simulink model "proposed"  (R2024b)
settings: Solver=VariableStepAuto  StartTime=0.0  StopTime=10  RelTol=1e-3
undefined symbols (not defined in the file or in its folder): G, Initial_level, IR, Qin_L, Qout_L, SA_U, TE, Temp, Water_Const, WD
libraries: spsVoltageMeasurementLib x10, spsSeriesRLCBranchLib x5, spsGroundLib x4, spsIGBTDiodeLib x4, simulink x3, spsThreePhaseParallelRLCLoadLib x2, spsCurrentMeasurementLib x2, spsPVArrayLib x2, spspowerguiLib x2, spsThreePhaseSourceLib x1, spsExcitationSystemLib x1, spsHydraulicTurbineandGovernorLib x1
settings Model: Creator=skill  LastModifiedBy=skill
settings DataIOCC: ReturnWorkspaceOutputs=off
settings OptimizationCC: DefaultUnderspecifiedDataType=single

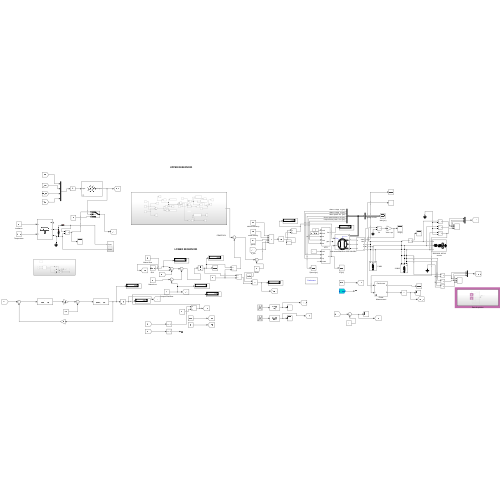
[thumbnail: Simulink's stored preview of the top-level diagram]
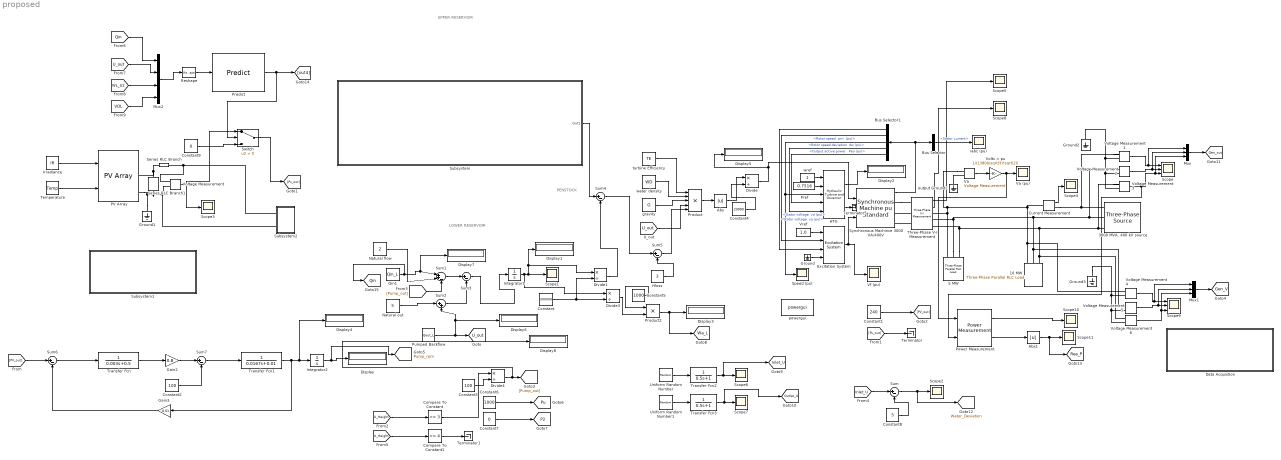
== system proposed ==
  note: UPPER RESERVOIR
  note: PENSTOCK
  note: LOWER RESERVOIR
  " Iabc (pu)" : Scope
  " Speed (pu)" : Scope
  10 MW : spsThreePhaseParallelRLCLoadLib/Three-Phase Parallel RLC Load  LConnTagsString=A|B|C  Configuration=Y (grounded)  NominalVoltage=400  Vabc=[1e3 1e3 1e3]  Vabcp=[1e3 1e3 1e3]  NominalFrequency=50  UnbalancedPower=off  ActivePower=360  InductivePower=0  CapacitivePower=0  Pabc=[10e3 9e3 11e3]  QLabc=[100 90 110]  QCabc=[100 90 110]  Pabcp=[10e3 9e3 11e3]  QLabcp=[100 90 110]  QCabcp=[100 90 110]  Measurements=None  LoadType=constant Z
  "3000 MVA, 400 kV source" : spsThreePhaseSourceLib/Three-Phase Source  InternalConnection=Yg  VoltagePhases=off  Voltage=400  PhaseAngle=0  Voltage_phases=[25e3 25e3 25e3]/sqrt(3)  PhaseAngles_phases=[0 -120 +120]  Frequency=50  NonIdealSource=on  SpecifyImpedance=on  Resistance=0.529  Inductance=0.0140  ShortCircuitLevel=3000  BaseVoltage=400  XRratio=10  BusType=swing  Pref=10e3  Qref=0  Prefabc=[10e3, 10e3, 10e3]  Qrefabc=[0, 0, 0]  Qmin=-inf  Qmax=inf
  5 MW : spsThreePhaseParallelRLCLoadLib/Three-Phase Parallel RLC Load  LConnTagsString=A|B|C  Configuration=Y (grounded)  NominalVoltage=380  Vabc=[1e3 1e3 1e3]  Vabcp=[1e3 1e3 1e3]  NominalFrequency=50  UnbalancedPower=off  ActivePower=200  InductivePower=0  CapacitivePower=0  Pabc=[10e3 9e3 11e3]  QLabc=[100 90 110]  QCabc=[100 90 110]  Pabcp=[10e3 9e3 11e3]  QLabcp=[100 90 110]  QCabcp=[100 90 110]  Measurements=None  LoadType=constant Z
  Abs : Abs  SaturateOnIntegerOverflow=off
  Abs1 : Abs  SaturateOnIntegerOverflow=off
  Bus Selector : BusSelector  OutputSignals=Stator current
  Bus Selector1 : BusSelector  OutputSignals="dq0 components.Stator voltage  vq (pu),dq0 components.Stator voltage  vd (pu),Mechanical.Rotor speed  wm  (pu),Mechanical.Rotor speed deviation  dw (pu),Output active power   Peo (pu)"
  Compare To Constant : simulink/Logic and Bit Operations/Compare To Constant  relop=<=  const=3  OutDataTypeStr=boolean
  Compare To Constant1 : simulink/Logic and Bit Operations/Compare To Constant  relop=>=  const=4  OutDataTypeStr=boolean
  Constant : Constant  Value=300000
  Constant1 : Constant  Value=240
  Constant2 : Constant  Value=100
  Constant3 : Constant  Value=100
  Constant4 : Constant  Value=23000
  Constant5 : Constant  Value=1000
  Constant6 : Constant  Value=1000
  Constant7 : Constant  Value=0
  Constant8 : Constant  Value=5
  Constant9 : Constant  Value=0
  Current Measurement : spsCurrentMeasurementLib/Current Measurement  PhasorSimulation=off  OutputType=Complex  PSBequivalent=0
  Data Acquistion : Subsystem
  Display{,1..8} (9 alike) : Display
  Divide{,1,3..4} (4 alike) : Product  Inputs=*/
  Excitation System : spsExcitationSystemLib/Excitation System  tr=20e-3  reg=[ 300, 0.001 ]  exc=[ 1, 0 ]  tgr=[ 0, 0 ]  damp=[ 0.001, 0.1 ]  sat=[ 0, 0 ]  lim=[ -11.5, 11.5, 0 ]  v0=[1,1.0]
  Gain2 : Gain  Gain=0.8
  Gain3 : Gain  Gain=0.01
  Ground : Ground
  Ground1 : spsGroundLib/Ground  LConnTagsString=a
  Ground2 : spsGroundLib/Ground  LConnTagsString=a
  Ground3 : spsGroundLib/Ground  LConnTagsString=a
  HTG : spsHydraulicTurbineandGovernorLib/Hydraulic Turbine and Governor  sm="[ 10/3  0.07 ]"  gate="[  0.01  0.97518  -0.1  0.1 ]"  reg="[  0.05  1.163  0.105  0  0.01  ]"  hyd="[  0  2.67  ]"  dref=0  po=1
  Hloss : Constant  Value=3
  Integrator1 : Integrator  InitialCondition=3000
  Integrator2 : Integrator  LimitOutput=on  UpperSaturationLimit=1500  LowerSaturationLimit=0
  Irradiance : Constant  Value=IR
  Mux : Mux  Inputs=3
  Mux1 : Mux  Inputs=3
  Mux2 : Mux
  Natural flow : Constant  Value=2
  Natural out : Constant  Value=5
  PV Array : spsPVArrayLib/PV Array  Npar=8  Nser=6  PlotType=array @ 1000 W/m2 & specified temperatures  S_vec="[ 1000  500  100 ]"  Temp_C_vec="[ 45 25  ]"  ModuleName=Vikram Solar Eldora VSP.60.240.03  PlotWhenSelected=off  Pm=242.489  Ncell=60  Voc=37.3  Isc=8.69  Vm=29.9  Im=8.11  beta_Voc_pc=-0.3426  alpha_Isc_pc=-0.012796  beta_Voc=-0.12779  alpha_Isc=-0.001112  IL=8.7088  I0=1.4122e-10  nI=0.9747  Rsh=212.3051  Rs=0.36536  RobustModel=off  RobustCellTemperature=313.3991  BAL=on  Tc=1e-6  Tfilter=5e-5
  Power Measurement : eePowerMeasurement/Power Measurement  LabelModeActiveChoice=Continuous  F=60  K=[0 1 2 3]  Ts=0
  Predict : deeplib/Predict  Network=Network from MAT-file  NetworkFunction=squeezenet  NetworkFilePath=D:\Ajay\Ajay-Electrical\2025\October\Brahma_nand_Thakur\Analysis\trained_deep_ANN.mat  MiniBatchSize=32  InputDataFormats={ '', '' }  Predictions=on  Activations={}  ForceInterpretedSim=off  EnableDLNetwork=on  LastKnownNetworkFilePath=''  LastKnownNetworkTimeStamp=''
  Pref : Constant  Value=0.7516
  Product : Product  Inputs=5
  Product2 : Product
  Pumped Backflow : Constant  Value=Qout_L
  Qin1 : Constant  Value=Qin_L
  Reshape : Reshape  OutputDimensionality=Customize  OutputDimensions=[1,4]
  Scope : Scope  NumInputPorts=3
  Scope{1..8,10..11} (10 alike) : Scope
  Scope9 : Scope  NumInputPorts=3
  Series RLC Branch : spsSeriesRLCBranchLib/Series RLC Branch  LConnTagsString=__new0  RConnTagsString=__new0  BranchType=R  Resistance=2  Inductance=1e-3  SetiL0=off  InitialCurrent=0  Capacitance=1e-6  Setx0=off  InitialVoltage=0  Measurements=None
  Series RLC Branch1 : spsSeriesRLCBranchLib/Series RLC Branch  LConnTagsString=__new0  RConnTagsString=__new0  BranchType=C  Resistance=1  Inductance=1e-3  SetiL0=off  InitialCurrent=0  Capacitance=1e-6  Setx0=off  InitialVoltage=0  Measurements=None
  Subsystem : Subsystem
  Subsystem1 : Subsystem
  Subsystem2 : Subsystem
  Sum{,3..7} (6 alike) : Sum  Inputs=|+-
  Sum1 : Sum  Inputs=|++-
  Sum2 : Sum  Inputs=|++
  Switch : Switch  Criteria=u2 > Threshold  SaturateOnIntegerOverflow=off  InputSameDT=off
  Synchronous Machince 3000 VA/400V : spsSynchronousMachinepuStandardLib/Synchronous Machine pu Standard  PresetModel=No  MechanicalLoad=Mechanical power Pm  ShowDetailedParameters=on  RotorType=Salient-pole  Units=per unit standard parameters  MeasurementBus=off  NominalParameters="[ 3000  400   50 ]"  Reactances1=[ 31 32 33 34 35 36 37 ]  Reactances2=[ 1.205, 0.196, 0.152, 0.374, 0.143, 0.08 ]  dAxisTimeConstants=Short-circuit  qAxisTimeConstants=Open-circuit  TimeConstants1=[]  TimeConstants2=[]  TimeConstants3=[]  TimeConstants4=[]  TimeConstants5=[ 1.01, 0.053, 0.1 ]  TimeConstants6=[]  TimeConstants7=[]  TimeConstants8=[]  StatorResistance=2.8544e-3  Mechanical="[ 3.2 0  32]"  PolePairs=32  InitialConditions=[0 0 0 0 0 0 0 0 1]  SetSaturation=off  Saturation=[0.6404,0.7127,0.8441,0.9214,0.9956,1.082,1.19,1.316,1.457;0.7,0.7698,0.8872,0.9466,0.9969,1.046,1.1,1.151,1.201]  LoadFlowParameters=[1 150000000 0 0]  TsPowergui=0  TsBlock=-1  IterativeModel=Forward Euler  IterativeDiscreteModel=Trapezoidal non iterative  BusType=PV  Pref=0  Qref=0  Qmin=-inf  Qmax=inf  PLF=0  QLF=0
  Temperature : Constant  Value=Temp
  Terminator : Terminator
  Terminator1 : Terminator
  Terminator5 : Terminator
  Three-Phase V-I Measurement : spsThreePhaseVIMeasurementLib/Three-Phase V-I Measurement  VoltageMeasurement=phase-to-ground  SetLabelV=off  LabelV=Vabc  Vpu=off  VpuLL=off  CurrentMeasurement=yes  SetLabelI=off  LabelI=Iabc  Ipu=off  Pbase=100e6  Vbase=500e3  OutputType=Complex  PhasorSimulation=off  PSBequivalent=0
  Transfer Fcn : TransferFcn  Denominator=[0.003 0.5]
  Transfer Fcn1 : TransferFcn  Denominator=[0.0167 0.01]
  Transfer Fcn2 : TransferFcn  Denominator=[0.5 1]
  Transfer Fcn3 : TransferFcn  Denominator=[0.5 1]
  Uniform Random Number : UniformRandomNumber  Minimum=8  Maximum=10  Seed=42  SampleTime=0.1
  Uniform Random Number1 : UniformRandomNumber  Minimum=10  Maximum=12  Seed=3  SampleTime=0.1
  Va : spsVoltageMeasurementLib/Voltage Measurement  Tag=PoWeRsYsTeMmEaSuReMeNt  PhasorSimulation=off  OutputType=Magnitude  PSBequivalent=0
  Va (pu) : Scope
  Vf (pu) : Scope
  Voltage Measurement{,1..6} (7 alike) : spsVoltageMeasurementLib/Voltage Measurement  PhasorSimulation=off  OutputType=Complex  PSBequivalent=0
  Volts > pu : Gain  Gain=1/(13800/sqrt(3)*sqrt(2))  SaturateOnIntegerOverflow=on  OutDataTypeStr=Inherit: Same as input  ParamDataTypeStr=Inherit: Same as input
  Vref : Constant  Value=1.0
  gravity : Constant  Value=G
  output Ground2 : spsGroundLib/Ground  LConnTagsString=a
  powergui : spspowerguiLib/powergui  Priority=2  SimulationMode=Continuous  SampleTime=0  frequency=60  Iterations=50  frequencyindice=50  Pbase=100e6  ErrMax=1e-4  UnitsV=kV  UnitsW=MW  buscounter=0  FunctionMessages=off  echomessages=off  EnableUseOfTLC=off  CurrentSourceSwitches=on  DisableSnubberDevices=off  DisableRonSwitches=off  DisableVfSwitches=off  DisplayEquations=off  AutomaticDiscreteSolvers=off  SolverType=Tustin/Backward Euler (TBE)  Interpol=off  ExternalGateDelay=off  methode=off  Ts=0  x0status=blocks  SPID=off  SwTol=0  HookPort=off  NonlinearTolerance=1e-4  nMaxIteration=100  ContinueOnMaxIteration=off  RestoreLinks=warning  ResistiveCurrentMeasurement=off  Frange=logspace(0,3,50)  Ylog=off  Xlog=off  ShowGrid=off  save=off  variable=ZData  structure=0  ZoomFFT=on  StartTime=0.0  cycles=2  DisplayStyle=off  fundamental=60  FreqAxis=off  MaxFrequency=1000  frequencyindicesteady=1  RmsSteady=1  display=off
  turbine Efficiency : Constant  Value=TE
  water density : Constant  Value=WD
  wref : Constant
  tag scope: Gen_V=global, Gen_out=global, Inlet_U=global, Outlet_U=global, P2=global, Pu=global, Pump_rpm=global, Qin=global, Rea_P=global, U_out=global, Wa_L=global, Water_Deviation=global
  wires:
  Constant5/1 -> Product2/1
  Constant6/1 -> [Pu]
  Constant7/1 -> [P2]
  Product2/1 -> [Wa_L], Display3/1
  Divide3/1 -> Product2/2
  Hloss/1 -> Sum5/2
  Constant3/1 -> Divide4/2
  Subsystem/1(Out1) -> Sum4/1
  Constant/1 -> Divide3/2, Divide1/2
  [Pv_out] -> Terminator/1
  Sum2/1 -> Sum3/2
  Constant1/1 -> [PV_out]
  Divide1/1 -> Sum4/2
  Sum3/1 -> Integrator1/1
  Natural out/1 -> Sum2/1
  Temperature/1 -> PV Array/2
  gravity/1 -> Product/3
  Voltage Measurement/1 -> Scope3/1, Switch/1
  Constant2/1 -> Sum7/2
  Transfer Fcn1/1 -> Display4/1, Integrator2/1, Gain3/1
  Sum4/1 -> Sum5/1
  Sum5/1 -> Product/5
  Product/1 -> Abs/1
  Transfer Fcn/1 -> Gain2/1
  [U_Height] -> Compare To Constant/1
  Gain3/1 -> Sum6/2
  [U_Height] -> Compare To Constant1/1
  [Pump_out] -> Sum1/3
  Irradiance/1 -> PV Array/1
  turbine Efficiency/1 -> Product/1
  water density/1 -> Product/2
  Integrator1/1 -> Divide3/1, Divide1/1, Display1/1, Scope1/1
  Sum1/1 -> Sum3/1
  Gain2/1 -> Sum7/1
  [PV_out] -> Sum6/1
  Sum6/1 -> Transfer Fcn/1
  Compare To Constant/1 -> Divide4/1
  Qin1/1 -> [Qin], Display7/1, Sum1/1
  Natural flow/1 -> Sum1/2
  Integrator2/1 -> [Pump_rpm], Display/1
  [U_out] -> Product/4
  Sum7/1 -> Transfer Fcn1/1
  Divide4/1 -> Display8/1, [Pump_out]
  Pumped Backflow/1 -> Display6/1, Sum2/2, [U_out]
  Compare To Constant1/1 -> Terminator1/1
  Bus Selector1/2 -> Excitation System/2  "<Stator voltage  vd (pu)>"
  HTG/2 -> Terminator5/1
  Ground/1 -> Excitation System/4
  wref/1 -> HTG/1
  Excitation System/1 -> Vf (pu)/1, Synchronous Machince 3000 VA/400V/2
  Bus Selector1/4 -> HTG/5  "<Rotor speed deviation  dw (pu)>"
  HTG/1 -> Display2/1
  Bus Selector1/1 -> Excitation System/3  "<Stator voltage  vq (pu)>"
  Pref/1 -> HTG/2
  Synchronous Machince 3000 VA/400V/1 -> Bus Selector/1, Bus Selector1/1
  Vref/1 -> Excitation System/1
  Va/1 -> Volts > pu/1
  Bus Selector1/3 -> HTG/3, " Speed (pu)"/1  "<Rotor speed  wm  (pu)>"
  Bus Selector/1 -> " Iabc (pu)"/1  "<Stator current>"
  Volts > pu/1 -> Power Measurement/1, Va (pu)/1
  Bus Selector1/5 -> HTG/4  "<Output active power   Peo (pu)>"
  Voltage Measurement1/1 -> Mux/1, Scope/1
  Voltage Measurement2/1 -> Mux/2, Scope/2
  Voltage Measurement3/1 -> Power Measurement/2, Mux/3, Scope/3
  Abs/1 -> Divide/1
  Constant4/1 -> Divide/2
  Three-Phase V-I Measurement/2 -> Scope8/1
  Three-Phase V-I Measurement/1 -> Scope5/1
  Uniform Random Number/1 -> Transfer Fcn2/1
  Transfer Fcn2/1 -> [Inlet_U], Scope6/1
  Transfer Fcn3/1 -> [Outlet_U], Scope7/1
  Uniform Random Number1/1 -> Transfer Fcn3/1
  Mux/1 -> [Gen_out]
  Mux1/1 -> [Gen_V]
  Voltage Measurement4/1 -> Mux1/1, Scope9/1
  Voltage Measurement6/1 -> Mux1/3, Scope9/3
  Voltage Measurement5/1 -> Mux1/2, Scope9/2
  [Inlet_U] -> Sum/1
  Constant8/1 -> Sum/2
  Current Measurement/1 -> Scope4/1
  Power Measurement/2 -> Abs1/1
  Abs1/1 -> [Rea_P], Scope11/1
  Sum/1 -> [Water_Deviation], Scope2/1
  Power Measurement/1 -> Scope10/1
  Divide/1 -> Synchronous Machince 3000 VA/400V/1, Display5/1
  [Qin] -> Mux2/1
  [U_out] -> Mux2/2
  [WL_U2] -> Mux2/3
  [VOL] -> Mux2/4
  Mux2/1 -> Reshape/1
  Reshape/1 -> Predict/1
  Predict/1 -> Switch/2, [out4]
  Constant9/1 -> Switch/3
  Switch/1 -> [Pv_out]
  connections:
  Ground1/LConn1 -- PV Array/RConn2 -- Subsystem2/LConn2 -- Voltage Measurement/LConn2 -- Series RLC Branch1/RConn1
  PV Array/RConn1 -- Series RLC Branch1/LConn1 -- Series RLC Branch/RConn1
  Voltage Measurement/LConn1 -- Series RLC Branch/LConn1 -- Subsystem2/LConn1
  5 MW/LConn2 -- Voltage Measurement5/LConn1 -- 10 MW/LConn2 -- Voltage Measurement2/LConn1 -- "3000 MVA, 400 kV source"/RConn2 -- Three-Phase V-I Measurement/RConn2
  5 MW/LConn3 -- Voltage Measurement6/LConn1 -- 10 MW/LConn3 -- Voltage Measurement3/LConn1 -- "3000 MVA, 400 kV source"/RConn3 -- Three-Phase V-I Measurement/RConn3
  Va/LConn1 -- Voltage Measurement4/LConn1 -- 10 MW/LConn1 -- Current Measurement/LConn1 -- 5 MW/LConn1 -- Three-Phase V-I Measurement/RConn1
  Synchronous Machince 3000 VA/400V/RConn1 -- Three-Phase V-I Measurement/LConn1
  output Ground2/LConn1 -- Va/LConn2
  Voltage Measurement1/LConn2 -- Voltage Measurement3/LConn2 -- Voltage Measurement2/LConn2 -- Ground2/LConn1
  Three-Phase V-I Measurement/LConn3 -- Synchronous Machince 3000 VA/400V/RConn3
  Three-Phase V-I Measurement/LConn2 -- Synchronous Machince 3000 VA/400V/RConn2
  Ground3/LConn1 -- Voltage Measurement4/LConn2 -- Voltage Measurement6/LConn2 -- Voltage Measurement5/LConn2
  Voltage Measurement1/LConn1 -- "3000 MVA, 400 kV source"/RConn1 -- Current Measurement/RConn1

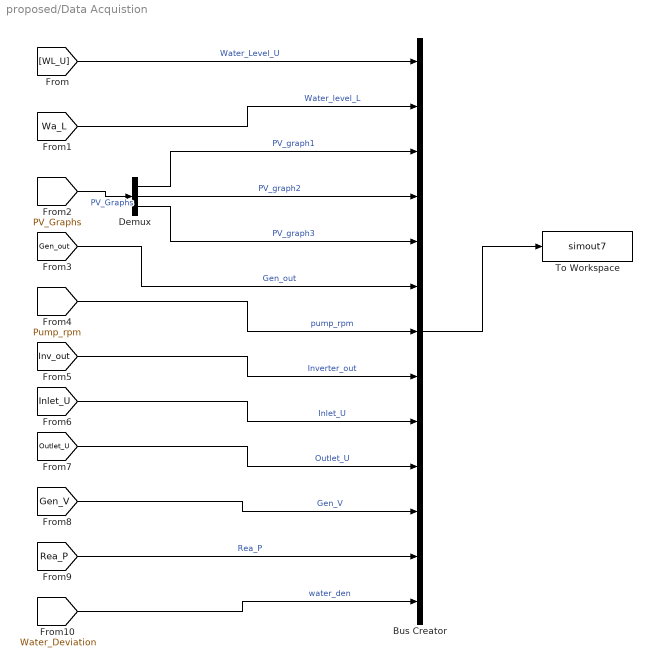
== system proposed/Data Acquistion ==
  Bus Creator : BusCreator  Inputs=13
  Demux : Demux  Outputs=3
  To Workspace : ToWorkspace  VariableName=simout7  SaveFormat=Timeseries  SampleTime=-1
  wires:
  Demux/3 -> Bus Creator/5  "PV_graph3"
  [Pump_rpm] -> Bus Creator/7  "pump_rpm"
  [Water_Deviation] -> Bus Creator/13  "water_den"
  Bus Creator/1 -> To Workspace/1
  [Inlet_U] -> Bus Creator/9  "Inlet_U"
  Demux/2 -> Bus Creator/4  "PV_graph2"
  [Gen_out] -> Bus Creator/6  "Gen_out"
  [Inv_out] -> Bus Creator/8  "Inverter_out"
  [PV_Graphs] -> Demux/1  "PV_Graphs"
  Demux/1 -> Bus Creator/3  "PV_graph1"
  [WL_U] -> Bus Creator/1  "Water_Level_U"
  [Outlet_U] -> Bus Creator/10  "Outlet_U"
  [Gen_V] -> Bus Creator/11  "Gen_V"
  [Rea_P] -> Bus Creator/12  "Rea_P"
  [Wa_L] -> Bus Creator/2  "Water_level_L"

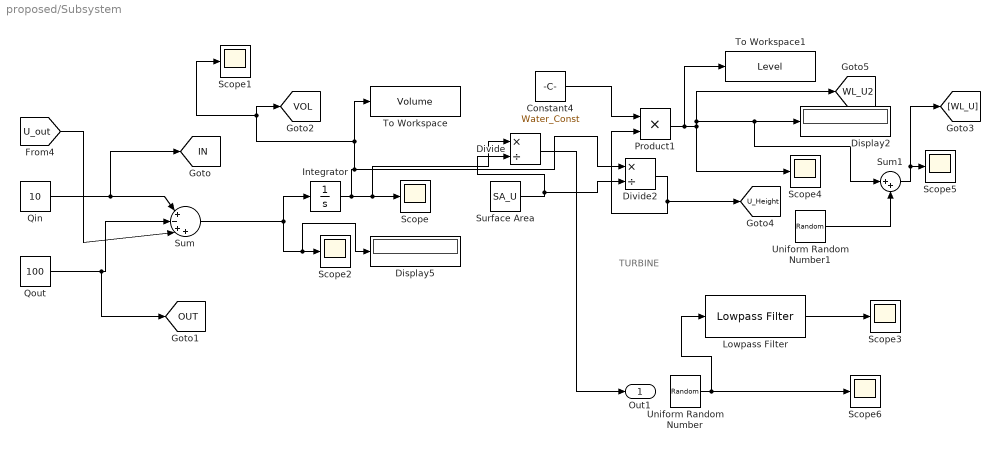
== system proposed/Subsystem ==
  note: TURBINE
  Constant4 : Constant  Value=Water_Const
  Display2 : Display
  Display5 : Display
  Divide : Product  Inputs=*/
  Divide2 : Product  Inputs=*/
  Integrator : Integrator  InitialCondition=Initial_level
  Lowpass Filter : dspfdesign/Lowpass Filter  FilterType=FIR  DesignForMinimumOrder=on  FilterOrder=50  PassbandFrequency=8e3  StopbandFrequency=12e3  PassbandRipple=0.1  StopbandAttenuation=80  SampleRateMode=Specify on dialog  SampleRate=44100  SimulateUsing=Interpreted execution  roundingMode=Floor  coeffsDataTypeStr=fixdt(1,16)
  Product1 : Product
  Qin : Constant  Value=10
  Qout : Constant  Value=100
  Scope{,1..6} (7 alike) : Scope
  Sum : Sum  Inputs=|+-++
  Sum1 : Sum  Inputs=|++
  Surface Area : Constant  Value=SA_U
  To Workspace : ToWorkspace  VariableName=Volume  SaveFormat=Timeseries  SampleTime=-1
  To Workspace1 : ToWorkspace  VariableName=Level  SaveFormat=Timeseries  SampleTime=-1
  Uniform Random Number : UniformRandomNumber  Minimum=9.6  Maximum=10  Seed=16  SampleTime=0.01
  Uniform Random Number1 : UniformRandomNumber  Minimum=-0.05  Maximum=0.05  SampleTime=0.1
  Out1 : Outport
  tag scope: IN=global, OUT=global, U_Height=global, VOL=global, WL_U2=global
  wires:
  Qin/1 -> [IN], Sum/1
  Constant4/1 -> Product1/1
  Integrator/1 -> Scope1/1, [VOL], To Workspace/1, Divide2/1, Divide/1, Scope/1
  Surface Area/1 -> Divide2/2, Divide/2
  Sum/1 -> Display5/1, Scope2/1, Integrator/1
  Divide2/1 -> [U_Height], Product1/2
  Qout/1 -> [OUT], Sum/2
  Product1/1 -> To Workspace1/1, [WL_U2], Sum1/1, Display2/1, Scope4/1
  Divide/1 -> Out1/1
  [U_out] -> Sum/3
  Uniform Random Number/1 -> Scope6/1, Lowpass Filter/1
  Lowpass Filter/1 -> Scope3/1
  Uniform Random Number1/1 -> Sum1/2
  Sum1/1 -> [WL_U], Scope5/1

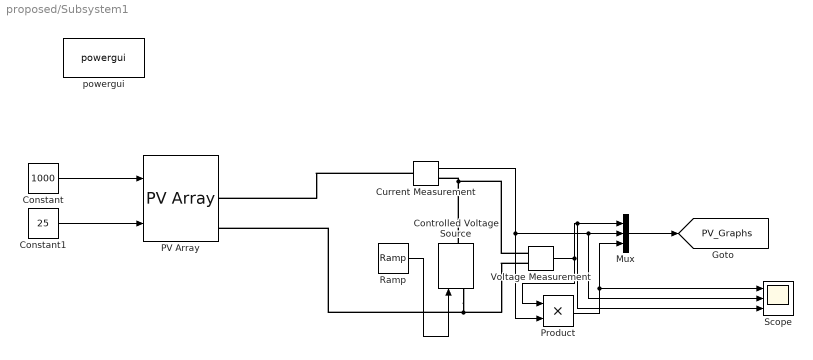
== system proposed/Subsystem1 ==
  Constant : Constant  Value=1000
  Constant1 : Constant  Value=25
  Controlled Voltage Source : spsControlledVoltageSourceLib/Controlled Voltage Source  Initialize=on  Source_Type=AC  Amplitude=0  Phase=0  Frequency=0  Measurements=None
  Current Measurement : spsCurrentMeasurementLib/Current Measurement  PhasorSimulation=off  OutputType=Complex  PSBequivalent=0
  Mux : Mux  Inputs=3
  PV Array : spsPVArrayLib/PV Array  Npar=1  Nser=9  PlotType=array @ 1000 W/m2 & specified temperatures  S_vec="[ 1000  500  100 ]"  Temp_C_vec="[ 45 25  ]"  ModuleName=User-defined  PlotWhenSelected=off  Pm=213.15  Ncell=60  Voc=36.3  Isc=7.84  Vm=29  Im=7.35  beta_Voc_pc=-0.36099  alpha_Isc_pc=0.102  beta_Voc=-0.13104  alpha_Isc=0.0079968  IL=7.8654  I0=2.9273e-10  nI=0.98119  Rsh=313.0553  Rs=0.39381  RobustModel=off  RobustCellTemperature=313.3991  BAL=on  Tc=1e-6  Tfilter=5e-5
  Product : Product
  Ramp : simulink/Sources/Ramp  slope=40  start=0  InitialOutput=0
  Scope : Scope  NumInputPorts=3
  Voltage Measurement : spsVoltageMeasurementLib/Voltage Measurement  PhasorSimulation=off  OutputType=Complex  PSBequivalent=0
  powergui : spspowerguiLib/powergui  Priority=1  SimulationMode=Continuous  SampleTime=50e-6  frequency=60  Iterations=50  frequencyindice=60  Pbase=100e6  ErrMax=1e-4  UnitsV=kV  UnitsW=MW  buscounter=0  FunctionMessages=off  echomessages=off  EnableUseOfTLC=off  CurrentSourceSwitches=off  DisableSnubberDevices=off  DisableRonSwitches=off  DisableVfSwitches=off  DisplayEquations=off  AutomaticDiscreteSolvers=off  SolverType=Tustin/Backward Euler (TBE)  Interpol=off  ExternalGateDelay=off  methode=off  Ts=100  x0status=blocks  SPID=on  SwTol=0  HookPort=off  NonlinearTolerance=1e-4  nMaxIteration=100  ContinueOnMaxIteration=off  RestoreLinks=warning  ResistiveCurrentMeasurement=off  Frange=[0:2:500]  Ylog=off  Xlog=on  ShowGrid=off  save=off  variable=ZData  structure=0  ZoomFFT=off  StartTime=0.0  cycles=1  DisplayStyle=1  fundamental=60  FreqAxis=off  MaxFrequency=1000  frequencyindicesteady=1  RmsSteady=1  display=off
  tag scope: PV_Graphs=global
  wires:
  Constant/1 -> PV Array/1
  Constant1/1 -> PV Array/2
  Ramp/1 -> Controlled Voltage Source/1
  Voltage Measurement/1 -> Product/1, Scope/3, Mux/1
  Current Measurement/1 -> Product/2, Scope/2, Mux/2
  Product/1 -> Mux/3, Scope/1
  Mux/1 -> [PV_Graphs]
  connections:
  Current Measurement/LConn1 -- PV Array/RConn1
  Current Measurement/RConn1 -- Controlled Voltage Source/RConn1 -- Voltage Measurement/LConn1
  PV Array/RConn2 -- Controlled Voltage Source/LConn1 -- Voltage Measurement/LConn2

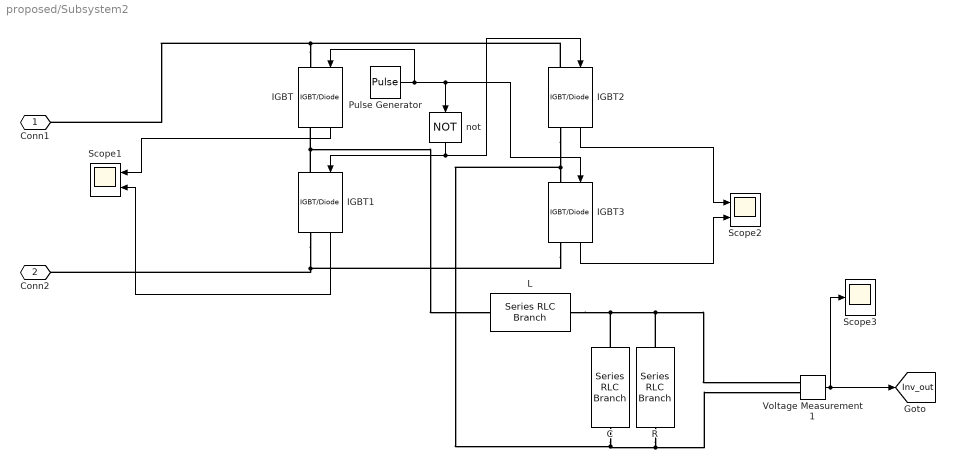
== system proposed/Subsystem2 ==
  " C" : spsSeriesRLCBranchLib/Series RLC Branch  LConnTagsString=__new0  RConnTagsString=__new0  BranchType=C  Resistance=1  Inductance=100e-3  SetiL0=off  InitialCurrent=0  Capacitance=470e-6  Setx0=off  InitialVoltage=450  Measurements=None
  " R" : spsSeriesRLCBranchLib/Series RLC Branch  LConnTagsString=__new0  RConnTagsString=__new0  BranchType=R  Resistance=10  Inductance=0.1  SetiL0=off  InitialCurrent=0  Capacitance=0  Setx0=off  InitialVoltage=0  Measurements=None
  IGBT{,1..3} (4 alike) : spsIGBTDiodeLib/IGBT//Diode  Ron=1e-3  Rs=1e5  Cs=inf  Measurements=on
  L : spsSeriesRLCBranchLib/Series RLC Branch  LConnTagsString=__new0  RConnTagsString=__new0  BranchType=L  Resistance=1  Inductance=36e-3  SetiL0=off  InitialCurrent=0  Capacitance=0  Setx0=off  InitialVoltage=0  Measurements=None
  Pulse Generator : DiscretePulseGenerator  PulseType=Time based  Period=0.02  PulseWidth=50
  Scope1 : Scope  NumInputPorts=2
  Scope2 : Scope  NumInputPorts=2
  Scope3 : Scope
  Voltage Measurement1 : spsVoltageMeasurementLib/Voltage Measurement  PhasorSimulation=off  OutputType=Complex  PSBequivalent=0
  not : Logic  Operator=NOT  AllPortsSameDT=off  OutDataTypeStr=boolean
  Conn1 : PMIOPort  Side=Left
  Conn2 : PMIOPort  Port=2  Side=Left
  tag scope: Inv_out=global
  wires:
  IGBT/1 -> Scope1/1
  Pulse Generator/1 -> IGBT3/1, not/1, IGBT/1
  IGBT2/1 -> Scope2/1
  not/1 -> IGBT2/1, IGBT1/1
  Voltage Measurement1/1 -> Scope3/1, [Inv_out]
  IGBT1/1 -> Scope1/2
  IGBT3/1 -> Scope2/2
  connections:
  L/LConn1 -- " C"/LConn1 -- " R"/LConn1 -- Voltage Measurement1/LConn1
  IGBT1/LConn1 -- L/RConn1 -- IGBT/RConn1
  IGBT3/RConn1 -- Conn2/RConn1 -- IGBT1/RConn1
  IGBT2/RConn1 -- " C"/RConn1 -- " R"/RConn1 -- Voltage Measurement1/LConn2 -- IGBT3/LConn1
  IGBT/LConn1 -- Conn1/RConn1 -- IGBT2/LConn1
